simulink model "gfm_datacenter_sil"  (R2018b)
settings: Solver=ode45  StartTime=0.0  StopTime=100  RelTol=1e-3
PreLoadFcn:
  | load_system('../simulink_reference_models/test_sequence_lib');
  | load_system('../simulink_reference_models/controls_element_lib');
InitFcn:
  | close all;
  | clear all;
  | clc;
  | 
  | close all;
  | clear all;
  | clc;
  | 
  | % frequency nominals
  | F_NOM = 60;
  | W_NOM = 2 * pi * F_NOM;
  | 
  | % base values relative to inverter
  | % --------------------------------
  | VLL_INV_NOM = 34.5e3;
  | P_INV_NOM = 5e6;
  | Q_INV_NOM = 2.5e6;
  | S_INV_NOM = sqrt(P_INV_NOM^2 + Q_INV_NOM^2);
  | 
  | I_INV_BASE = S_INV_NOM/(sqrt(3)*VLL_INV_NOM);
  | Z_INV_BASE = VLL_INV_NOM^2/S_INV_NOM;
  | L_INV_BASE = Z_INV_BASE / W_NOM;
  | C_INV_BASE = 1 / (Z_INV_BASE * W_NOM);
  | 
  | % SST Parameters
  | N_DCDC_XFMR = 3;
  | N_CELLS_PER_STRING = 10;
  | C_MV_CELL = 400e-6;
  | C_LV_SST = 5e-3;
  | C_BBU = 1500; % 60 sec * 5MW
  | r_BBU = 5e-3;
  | ILV_MAX = 300;
  | ILV_MIN = -300;
  | IMV_MAX = 100;
  | IMV_MIN = -100;
  | V_LVDC_NOM = 800;
  | IDC_NOM = P_INV_NOM / V_LVDC_NOM;
  | 
  | % nominal ratings for power system model
  | % --------------------------------------
  | INVERTER_COUNT = 20;
  | 
  | VMV_NOM = VLL_INV_NOM;
  | VHV_NOM = 230e3;
  | S_PLANT = INVERTER_COUNT * S_INV_NOM;
  | 
  | N_GSU = VHV_NOM/VMV_NOM;
  | 
  | I_MV_BASE = S_PLANT/(sqrt(3)*VMV_NOM);
  | I_HV_BASE = S_PLANT/(sqrt(3)*VHV_NOM);
  | 
  | Z_MV_BASE = VMV_NOM^2/S_PLANT;
  | Z_HV_BASE = VHV_NOM^2/S_PLANT;
  | 
  | L_MV_BASE = Z_MV_BASE / W_NOM;
  | L_HV_BASE = Z_HV_BASE / W_NOM;
  | C_MV_BASE = 1 / (Z_MV_BASE * W_NOM);
  | C_HV_BASE = 1 / (Z_HV_BASE * W_NOM);
libraries: test_sequence_lib x14, controls_element_lib x3
settings Model: SimulationMode=accelerator  Creator=HussamAlatrash  LastModifiedBy=ahhei
settings DataIOCC: ReturnWorkspaceOutputs=on
settings DebuggingCC: UnconnectedInputMsg=none  UnconnectedOutputMsg=none  UnconnectedLineMsg=none
settings ModelReferenceCC: EnableRefExpFcnMdlSchedulingChecks=off
settings RTWCC: Description=Generic Real-Time Target
settings ConfigComp: CovBoundaryAbsTol=1.0e-5

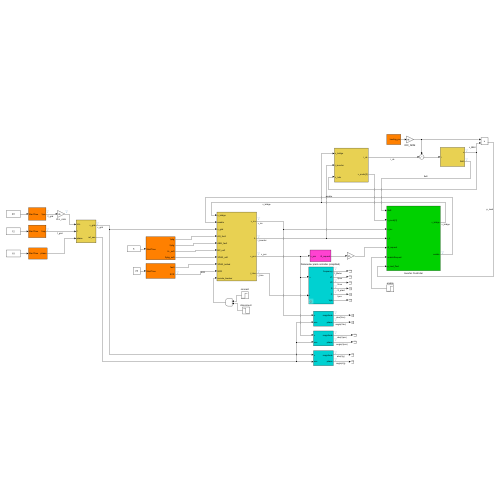
[thumbnail: Simulink's stored preview of the top-level diagram]
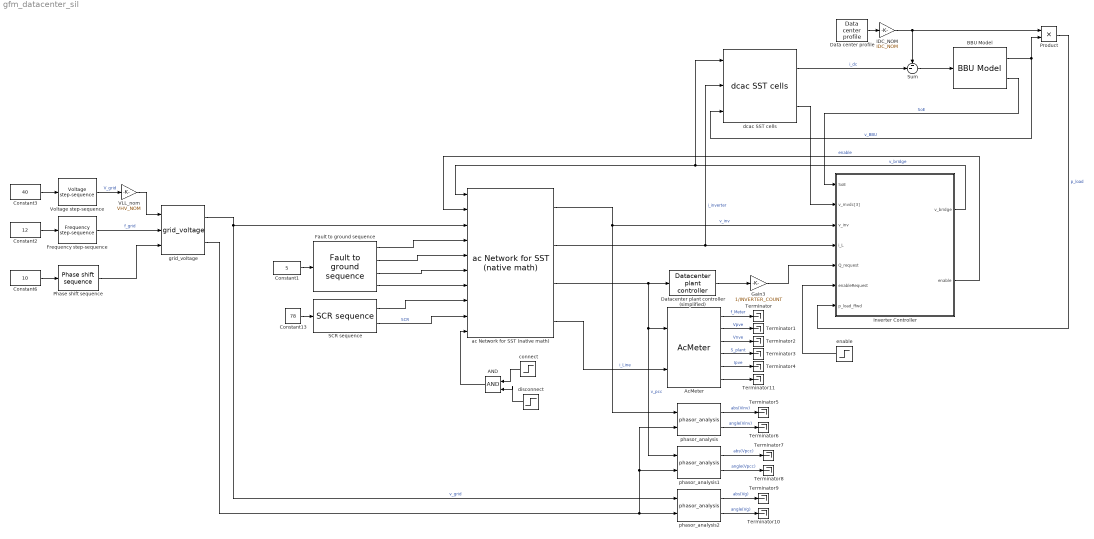
== system gfm_datacenter_sil ==
  AND : Logic  IconShape=distinctive  AllPortsSameDT=off  OutDataTypeStr=boolean
  AcMeter : test_sequence_lib/AcMeter  VllRated=VHV_NOM
  BBU Model : test_sequence_lib/BBU Model  SystemSampleTime=-1  EmptyChoice=off  PassThrough=off  PassThroughVariantControl=(default)  EmptyChoiceVariantControl=(default)  Latency=0  AutoFrameSizeCalculation=off
  Constant1 : Constant  Value=5
  Constant13 : Constant  Value=78
  Constant2 : Constant  Value=12
  Constant3 : Constant  Value=40
  Constant6 : Constant  Value=10
  Data center profile : test_sequence_lib/Data center profile  SystemSampleTime=-1  EmptyChoice=off  PassThrough=off  PassThroughVariantControl=(default)  EmptyChoiceVariantControl=(default)  Latency=0  AutoFrameSizeCalculation=off
  Datacenter plant controller (simplified) : controls_element_lib/Datacenter plant controller  SystemSampleTime=-1  EmptyChoice=off  PassThrough=off  PassThroughVariantControl=(default)  EmptyChoiceVariantControl=(default)  Latency=0  AutoFrameSizeCalculation=off
  Fault to ground sequence : test_sequence_lib/Fault to ground sequence  SystemSampleTime=-1  EmptyChoice=off  PassThrough=off  PassThroughVariantControl=(default)  EmptyChoiceVariantControl=(default)  Latency=0  AutoFrameSizeCalculation=off
  Frequency step-sequence : test_sequence_lib/Frequency step-sequence  SystemSampleTime=-1  EmptyChoice=off  PassThrough=off  PassThroughVariantControl=(default)  EmptyChoiceVariantControl=(default)  Latency=0  AutoFrameSizeCalculation=off
  Gain3 : Gain  Gain=1/INVERTER_COUNT
  IDC_NOM : Gain  Gain=IDC_NOM
  Inverter Controller : Subsystem
  Phase shift sequence : test_sequence_lib/Phase shift sequence  SystemSampleTime=-1  EmptyChoice=off  PassThrough=off  PassThroughVariantControl=(default)  EmptyChoiceVariantControl=(default)  Latency=0  AutoFrameSizeCalculation=off
  Product : Product
  SCR sequence : test_sequence_lib/SCR sequence  SystemSampleTime=-1  EmptyChoice=off  PassThrough=off  PassThroughVariantControl=(default)  EmptyChoiceVariantControl=(default)  Latency=0  AutoFrameSizeCalculation=off
  Sum : Sum  Inputs=--|
  Terminator{,1..11} (12 alike) : Terminator
  VLL_nom : Gain  Gain=VHV_NOM
  Voltage step-sequence : test_sequence_lib/Voltage step-sequence  SystemSampleTime=-1  EmptyChoice=off  PassThrough=off  PassThroughVariantControl=(default)  EmptyChoiceVariantControl=(default)  Latency=0  AutoFrameSizeCalculation=off
  ac Network for SST (native math) : test_sequence_lib/ac Network for SST (native math)  SystemSampleTime=-1  EmptyChoice=off  PassThrough=off  PassThroughVariantControl=(default)  EmptyChoiceVariantControl=(default)  Latency=0  AutoFrameSizeCalculation=off
  connect : Step  Time=0  SampleTime=0
  dcac SST cells : test_sequence_lib/dcac SST cells  SystemSampleTime=-1  EmptyChoice=off  PassThrough=off  PassThroughVariantControl=(default)  EmptyChoiceVariantControl=(default)  Latency=0  AutoFrameSizeCalculation=off
  disconnect : Step  Time=97  Before=1  After=0  SampleTime=0
  enable : Step  Time=2  SampleTime=0
  grid_voltage : test_sequence_lib/grid_voltage  SystemSampleTime=-1  EmptyChoice=off  PassThrough=off  PassThroughVariantControl=(default)  EmptyChoiceVariantControl=(default)  Latency=0  AutoFrameSizeCalculation=off
  phasor_analysis : test_sequence_lib/phasor_analysis  SystemSampleTime=-1  EmptyChoice=off  PassThrough=off  PassThroughVariantControl=(default)  EmptyChoiceVariantControl=(default)  Latency=0  AutoFrameSizeCalculation=off
  phasor_analysis1 : test_sequence_lib/phasor_analysis  SystemSampleTime=-1  EmptyChoice=off  PassThrough=off  PassThroughVariantControl=(default)  EmptyChoiceVariantControl=(default)  Latency=0  AutoFrameSizeCalculation=off
  phasor_analysis2 : test_sequence_lib/phasor_analysis  SystemSampleTime=-1  EmptyChoice=off  PassThrough=off  PassThroughVariantControl=(default)  EmptyChoiceVariantControl=(default)  Latency=0  AutoFrameSizeCalculation=off
  wires:
  phasor_analysis/1 -> Terminator5/1  "abs(Vinv)"
  AcMeter/6 -> Terminator11/1
  Product/1 -> Inverter Controller/7(p_load_ffwd)  "p_load"
  Constant3/1 -> Voltage step-sequence/1
  SCR sequence/1 -> ac Network for SST (native math)/8
  Fault to ground sequence/3 -> ac Network for SST (native math)/6
  Data center profile/1 -> IDC_NOM/1
  SCR sequence/2 -> ac Network for SST (native math)/9  "SCR"
  AcMeter/1 -> Terminator/1  "f_Meter"
  Datacenter plant controller (simplified)/1 -> Gain3/1
  AcMeter/5 -> Terminator4/1  "Ipve"
  VLL_nom/1 -> grid_voltage/1
  AcMeter/3 -> Terminator2/1  "Vnve"
  phasor_analysis1/1 -> Terminator7/1  "abs(Vpcc)"
  Inverter Controller/1(v_bridge) -> dcac SST cells/1, ac Network for SST (native math)/1  "v_bridge"
  Constant1/1 -> Fault to ground sequence/1
  phasor_analysis2/1 -> Terminator9/1  "abs(Vg)"
  IDC_NOM/1 -> Sum/1, Product/1
  grid_voltage/1 -> ac Network for SST (native math)/3, phasor_analysis2/1  "v_grid"
  Frequency step-sequence/1 -> grid_voltage/2  "f_grid"
  enable/1 -> Inverter Controller/6(enableRequest)
  Sum/1 -> BBU Model/1
  phasor_analysis/2 -> Terminator6/1  "angle(Vinv)"
  BBU Model/2 -> Inverter Controller/1(SoE)  "SoE"
  AND/1 -> ac Network for SST (native math)/10
  ac Network for SST (native math)/1 -> phasor_analysis/1, Inverter Controller/3(v_inv)  "v_inv"
  Phase shift sequence/1 -> grid_voltage/3
  Fault to ground sequence/2 -> ac Network for SST (native math)/5
  phasor_analysis2/2 -> Terminator10/1  "angle(Vg)"
  ac Network for SST (native math)/4 -> AcMeter/2  "i_Line"
  Fault to ground sequence/1 -> ac Network for SST (native math)/4
  Constant2/1 -> Frequency step-sequence/1
  Voltage step-sequence/1 -> VLL_nom/1  "V_grid"
  grid_voltage/2 -> phasor_analysis1/2, phasor_analysis/2, phasor_analysis2/2
  ac Network for SST (native math)/3 -> Datacenter plant controller (simplified)/1, phasor_analysis1/1, AcMeter/1  "v_pcc"
  phasor_analysis1/2 -> Terminator8/1  "angle(Vpcc)"
  Fault to ground sequence/4 -> ac Network for SST (native math)/7
  dcac SST cells/1 -> Sum/2  "i_dc"
  dcac SST cells/2 -> Inverter Controller/2(v_mvdc[3])
  connect/1 -> AND/1
  BBU Model/1 -> dcac SST cells/3, Product/2  "v_BBU"
  AcMeter/4 -> Terminator3/1  "S_plant"
  AcMeter/2 -> Terminator1/1  "Vpve"
  Constant13/1 -> SCR sequence/1
  ac Network for SST (native math)/2 -> dcac SST cells/2, Inverter Controller/4(i_L)  "i_inverter"
  Constant6/1 -> Phase shift sequence/1
  disconnect/1 -> AND/2
  Gain3/1 -> Inverter Controller/5(Q_request)
  Inverter Controller/2(enable) -> ac Network for SST (native math)/2  "enable"

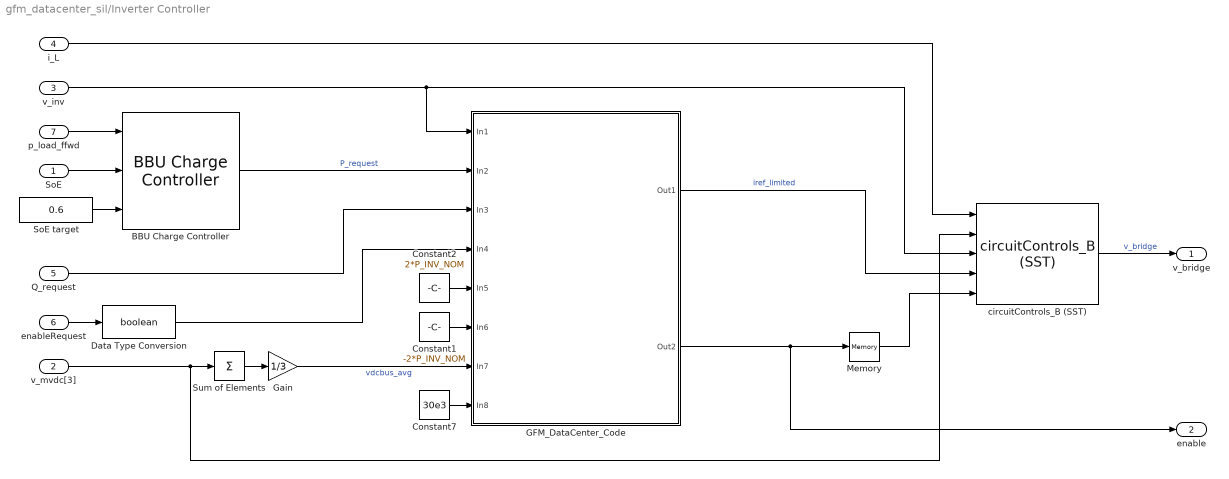
== system gfm_datacenter_sil/Inverter Controller ==
  SoE : Inport
  v_mvdc[3] : Inport  Port=2
  v_inv : Inport  Port=3
  i_L : Inport  Port=4
  Q_request : Inport  Port=5
  enableRequest : Inport  Port=6
  p_load_ffwd : Inport  Port=7
  BBU Charge Controller : controls_element_lib/BBU Charge Controller  SystemSampleTime=-1  EmptyChoice=off  PassThrough=off  PassThroughVariantControl=(default)  EmptyChoiceVariantControl=(default)  Latency=0  AutoFrameSizeCalculation=off
  Constant1 : Constant  Value=-2*P_INV_NOM
  Constant2 : Constant  Value=2*P_INV_NOM
  Constant7 : Constant  Value=30e3
  Data Type Conversion : DataTypeConversion  OutDataTypeStr=boolean
  GFM_DataCenter_Code : Subsystem  Description=Replaced Block  mask(Replaced Block){}
      mask help: This block has been replaced with an empty subsystem because it used functionality that is unavailable in Simulink R2018b.
      mask Display: fprintf('Replaced: %s\n','CFunction')
  Gain : Gain  Gain=1/3
  Memory : Memory
  SoE target : Constant  Value=0.6
  Sum of Elements : Sum  Inputs=+
  circuitControls_B (SST) : controls_element_lib/circuitControls_B (SST)  SystemSampleTime=-1  EmptyChoice=off  PassThrough=off  PassThroughVariantControl=(default)  EmptyChoiceVariantControl=(default)  Latency=0  AutoFrameSizeCalculation=off
  v_bridge : Outport
  enable : Outport  Port=2
  wires:
  GFM_DataCenter_Code/1(Out1) -> circuitControls_B (SST)/4  "iref_limited"
  Constant1/1 -> GFM_DataCenter_Code/6(In6)
  BBU Charge Controller/1 -> GFM_DataCenter_Code/2(In2)  "P_request"
  v_inv/1 -> circuitControls_B (SST)/3, GFM_DataCenter_Code/1(In1)
  Gain/1 -> GFM_DataCenter_Code/7(In7)  "vdcbus_avg"
  Constant7/1 -> GFM_DataCenter_Code/8(In8)
  circuitControls_B (SST)/1 -> v_bridge/1  "v_bridge"
  i_L/1 -> circuitControls_B (SST)/1
  Memory/1 -> circuitControls_B (SST)/5
  p_load_ffwd/1 -> BBU Charge Controller/1
  SoE/1 -> BBU Charge Controller/2
  SoE target/1 -> BBU Charge Controller/3
  Sum of Elements/1 -> Gain/1
  v_mvdc[3]/1 -> circuitControls_B (SST)/2, Sum of Elements/1
  Constant2/1 -> GFM_DataCenter_Code/5(In5)
  Q_request/1 -> GFM_DataCenter_Code/3(In3)
  GFM_DataCenter_Code/2(Out2) -> enable/1, Memory/1
  enableRequest/1 -> Data Type Conversion/1
  Data Type Conversion/1 -> GFM_DataCenter_Code/4(In4)

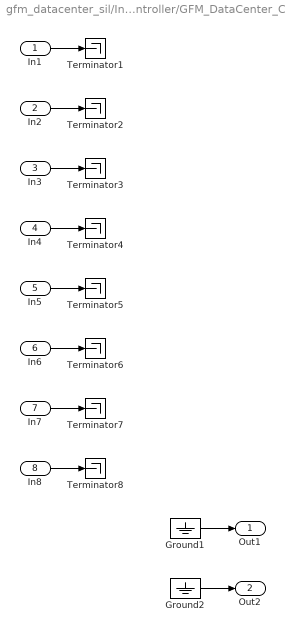
== system gfm_datacenter_sil/Inverter Controller/GFM_DataCenter_Code ==
  In1 : Inport
  In2 : Inport  Port=2
  In3 : Inport  Port=3
  In4 : Inport  Port=4
  In5 : Inport  Port=5
  In6 : Inport  Port=6
  In7 : Inport  Port=7
  In8 : Inport  Port=8
  Ground1 : Ground
  Ground2 : Ground
  Terminator{1..8} (8 alike) : Terminator
  Out1 : Outport
  Out2 : Outport  Port=2
  wires:
  Ground2/1 -> Out2/1
  Ground1/1 -> Out1/1
  In8/1 -> Terminator8/1
  In7/1 -> Terminator7/1
  In6/1 -> Terminator6/1
  In5/1 -> Terminator5/1
  In4/1 -> Terminator4/1
  In3/1 -> Terminator3/1
  In2/1 -> Terminator2/1
  In1/1 -> Terminator1/1
